simulink model "TECM_SeriesParallel"  (R2023a)
settings: Solver=daessc  StartTime=0.0  StopTime=20E4
libraries: fl_lib x34, nesl_utility x24, BatteryLibrary_lib x5
settings Model: Creator=widana_d  LastModifiedBy=widana_d
settings SolverCC: SolverResetMethod=Robust
settings DataIOCC: SaveState=on
settings OptimizationCC: ReuseModelBlockBuffer=off
settings DebuggingCC: UnconnectedInputMsg=warning  UnconnectedOutputMsg=warning  UnconnectedLineMsg=warning
settings ModelReferenceCC: EnableRefExpFcnMdlSchedulingChecks=on
settings RTWCC: DLArmComputeVersion=19.05

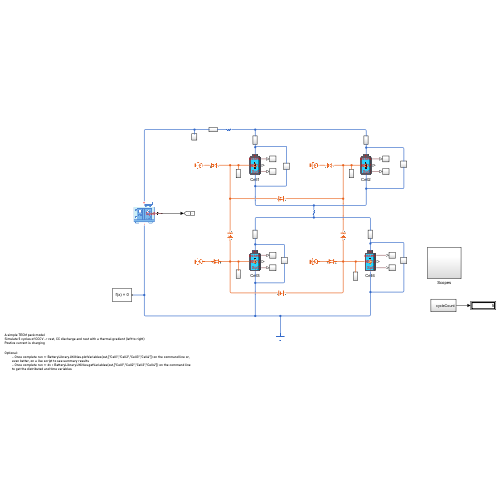
[thumbnail: Simulink's stored preview of the top-level diagram]
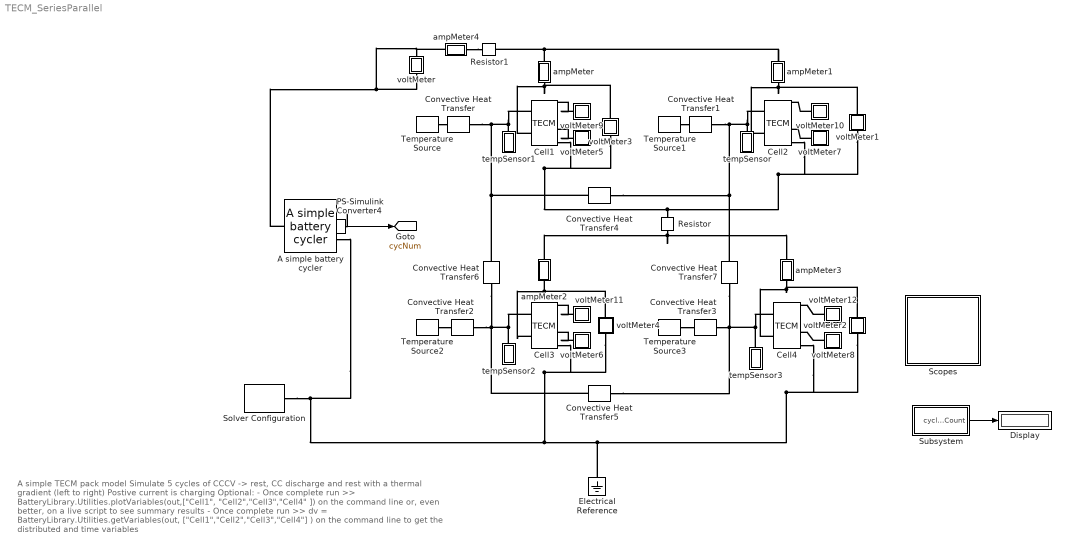
== system TECM_SeriesParallel ==
  note: A simple TECM pack model
      | Simulate 5 cycles of CCCV -> rest, CC discharge and rest with a thermal gradient (left to right)
      | Postive current is charging
      |
      | Optional:
      | - Once complete run >> BatteryLibrary.Utilities.plotVariables(out,["Cell1", "Cell2","Cell3","Cell4" ]) on the command line or, even better, on a live script to see summary results
      | - Once complete run >> dv = BatteryLibrary.Utilities.getVariables(out, ["Cell1","Cell2","Cell3","Cell4"] ) on the command line to get the distributed and time variables
  A simple battery cycler : BatteryLibrary_lib/Utilities/A simple battery cycler  Vmax=8.3 V  Vmin=6.2 V  Ic=4 A  Ico=0.5 A  Id=-10 A  tRestC=1800 s  tRestD=3600 s
      settings: InternalSimscapePortConfiguration="{\"Bottom\":[{\"id\":\"n\",\"label\":\"-\",\"type\":\"foundation.electrical.electrical\"}],\"Left\":[],\"Right\":[{\"id\":\"numCyc\",\"label\":\"Cyc#\",\"type\":\"output\"}],\"Top\":[{\"id\":\"p\",\"label\":\"+\",\"type\":\"foundation.electrical.electrical\"}]}"
  Cell{1..4} (4 alike) : BatteryLibrary_lib/Models/TECM  z0=0.2  T0=298 K  Cn=4.0 A*hr  RoLUT=[.116, .097, .0979, .111; .079, .0617, .0636, .0708; .0526, .0424, .0438, .0483; .0339, .0314, .0325, .0338] Ohm  RpLUT=[.153, .035, .0738, .051; .043, .0323, .0532, .0401; .0293, .0197, .0357, .021; .0124, .00855, .0183, .00974] Ohm  TauLUT=[3.42, 38.3, 66.8, 38.5; 3.19, 46.9, 59.6, 37.5; 47.1, 41.3, 63.9, 32; 23.2, 19.6, 41.2, 16.1] s  tempLUT=[273, 283, 298, 318] K  socLUT=[20.79, 50.5, 80.2, 95.05]/100  Cp=100 J/K  refSoC=[0 : 100]' / 100  refOCV=[3.32, 3.33, 3.34, 3.35, 3.35, 3.36, 3.38, 3.39, 3.4, 3.42, 3.43, 3.44, 3.45, 3.46, 3.47, 3.48, 3.49, 3.5, 3.51, 3.52, 3.52, 3.53, 3.54, 3.54, 3.55, 3.55, 3.56, 3.56, 3.57, 3.57, 3.58, 3.58, 3.59, 3.59, 3.6, 3.6, 3.61, 3.61, 3.62, 3.62, 3.63, 3.63, 3.64, 3.64, 3.65, 3.65, 3.66, 3.67, 3.68, 3.69, 3.7, 3.71, 3.72, 3.74, 3.75, 3.76, 3.76, 3.77, 3.78, 3.79, 3.8, 3.81, 3.81, 3.82, 3.83, 3.84, 3.85, 3.85, 3.86, 3.87, 3.88, 3.88, 3.89, 3.9, 3.9, 3.91, 3.92, 3.93, 3.94, 3.94, 3.95, 3.96, 3.97, 3.98, 3.99, 4, 4.01, 4.02, 4.03, 4.04, 4.05, 4.06, 4.07, 4.08, 4.09, 4.1, 4.11, 4.12, 4.13, 4.14, 4.15]' V
      settings: InternalSimscapePortConfiguration="{\"Bottom\":[{\"id\":\"n\",\"label\":\"-\",\"type\":\"foundation.electrical.electrical\"}],\"Left\":[{\"id\":\"Hi\",\"label\":\"H\",\"type\":\"foundation.thermal.thermal\"}],\"Right\":[{\"id\":\"eta\",\"label\":\"Losses\",\"type\":\"output\"},{\"id\":\"OCV\",\"label\":\"OCV\",\"type\":\"output\"},{\"id\":\"z\",\"label\":\"SoC\",\"type\":\"output\"}],\"Top\":[{\"id\":\"p\",\"label\":\"+\",\"type\":\"foundation.electrical.electrical\"}]}"
  Convective Heat Transfer{,1..3} (4 alike) : fl_lib/Thermal/Thermal Elements/Convective Heat Transfer  thermal_type=foundation.enum.constant_variable.constant  area=0.0023 m^2  heat_tr_coeff=35 W/(m^2 * K)  min_heat_tr_coeff=1e-3 W/(K*m^2)  T_specify=off  T_priority=None  T=0 K  T_nominal_specify=off  T_nominal_unit=K  T_nominal_value=1  Q_specify=off  Q_priority=None  Q=0 W  Q_nominal_specify=off  Q_nominal_unit=W  Q_nominal_value=1
  Convective Heat Transfer4 : fl_lib/Thermal/Thermal Elements/Convective Heat Transfer  thermal_type=foundation.enum.constant_variable.constant  area=0.0015 m^2  heat_tr_coeff=10 W/(m^2 * K)  min_heat_tr_coeff=1e-3 W/(K*m^2)  T_specify=off  T_priority=None  T=0 K  T_nominal_specify=off  T_nominal_unit=K  T_nominal_value=1  Q_specify=off  Q_priority=None  Q=0 W  Q_nominal_specify=off  Q_nominal_unit=W  Q_nominal_value=1
  Convective Heat Transfer5 : fl_lib/Thermal/Thermal Elements/Convective Heat Transfer  thermal_type=foundation.enum.constant_variable.constant  area=0.00115 m^2  heat_tr_coeff=10 W/(m^2 * K)  min_heat_tr_coeff=1e-3 W/(K*m^2)  T_specify=off  T_priority=None  T=0 K  T_nominal_specify=off  T_nominal_unit=K  T_nominal_value=1  Q_specify=off  Q_priority=None  Q=0 W  Q_nominal_specify=off  Q_nominal_unit=W  Q_nominal_value=1
  Convective Heat Transfer6 : fl_lib/Thermal/Thermal Elements/Convective Heat Transfer  thermal_type=foundation.enum.constant_variable.constant  area=0.00115 m^2  heat_tr_coeff=10 W/(m^2 * K)  min_heat_tr_coeff=1e-3 W/(K*m^2)  T_specify=off  T_priority=None  T=0 K  T_nominal_specify=off  T_nominal_unit=K  T_nominal_value=1  Q_specify=off  Q_priority=None  Q=0 W  Q_nominal_specify=off  Q_nominal_unit=W  Q_nominal_value=1
  Convective Heat Transfer7 : fl_lib/Thermal/Thermal Elements/Convective Heat Transfer  thermal_type=foundation.enum.constant_variable.constant  area=0.00115 m^2  heat_tr_coeff=10 W/(m^2 * K)  min_heat_tr_coeff=1e-3 W/(K*m^2)  T_specify=off  T_priority=None  T=0 K  T_nominal_specify=off  T_nominal_unit=K  T_nominal_value=1  Q_specify=off  Q_priority=None  Q=0 W  Q_nominal_specify=off  Q_nominal_unit=W  Q_nominal_value=1
  Display : Display
  Electrical Reference : fl_lib/Electrical/Electrical Elements/Electrical Reference
  PS-Simulink Converter4 : nesl_utility/PS-Simulink Converter  PhysicalDomain=network_engine_domain  SubClassName=ps_output  LeftPortType=input  RightPortType=output  PseudoPeriodic=off  Frequencies=[]  VectorFormat=1-D array  Unit=inherit  AffineConversion=off
  Resistor : fl_lib/Electrical/Electrical Elements/Resistor  R=1e-3 Ohm  i_specify=off  i_priority=None  i=0 A  i_nominal_specify=off  i_nominal_unit=A  i_nominal_value=1  v_specify=off  v_priority=None  v=0 V  v_nominal_specify=off  v_nominal_unit=V  v_nominal_value=1
  Resistor1 : fl_lib/Electrical/Electrical Elements/Resistor  R=1e-3 Ohm  i_specify=off  i_priority=None  i=0 A  i_nominal_specify=off  i_nominal_unit=A  i_nominal_value=1  v_specify=off  v_priority=None  v=0 V  v_nominal_specify=off  v_nominal_unit=V  v_nominal_value=1
  Scopes : Subsystem
  Solver Configuration : nesl_utility/Solver Configuration  PhysicalDomain=network_engine_domain  SubClassName=solver  LeftPortType=input  RightPortType=generic  Tones=[]  Harmonics=[]  SimulateNoise=off  Profile=off  UseLocalSampling=off  EnableSwitchedLinearOptims=on  FrequencyDomain=off  UseCCode=off  RelTol=0.001  AbsTol=1e-06  MinStep=1e-09  ToWorkspace=off  RevertToSquareIcSolve=off  NumHomotopyIterations=100  PhasorMode=off  PhasorModeNumHarmonics=1  ConsistencySolver=NEWTON_FTOL  IndexReductionMethod=DerivativeReplacement  DoDC=off  ResidualTolerance=1e-09  ConsistencyTolSource=GLOBAL  ConsistencyAbsTol=0.001  ConsistencyRelTol=0.001  ConsistencyTolFactor=0.001  UseLocalSolver=off  LocalSolverChoice=NE_BACKWARD_EULER_ADVANCER  ResolveIndetEquations=on  FunctionEvalNumThread=1  LocalSolverSampleTime=0.001  DoFixedCost=off  MaxNonlinIter=3  MaxModeIter=2  ComputeImpulses=off  ImpulseIterations=2  LinearAlgebra=auto  LinearAlgebraNumThread=0  EquationFormulation=NE_TIME_EF  DelaysMemoryBudget=1024  AutomaticFiltering=on  FilteringTimeConstant=0.001  PartitionStorageMethod=AS_NEEDED  PartitionMemoryBudget=1024  PartitionMethod=ROBUST
  Subsystem : Subsystem
  Temperature Source : fl_lib/Thermal/Thermal Sources/Temperature Source  temperature=20 degC
  Temperature Source1 : fl_lib/Thermal/Thermal Sources/Temperature Source  temperature=30 degC
  Temperature Source2 : fl_lib/Thermal/Thermal Sources/Temperature Source  temperature=20 degC
  Temperature Source3 : fl_lib/Thermal/Thermal Sources/Temperature Source  temperature=30 degC
  ampMeter : Subsystem
  ampMeter1 : Subsystem
  ampMeter2 : Subsystem
  ampMeter3 : Subsystem
  ampMeter4 : Subsystem
  tempSensor : Subsystem
  tempSensor1 : Subsystem
  tempSensor2 : Subsystem
  tempSensor3 : Subsystem
  voltMeter : Subsystem
  voltMeter1 : Subsystem
  voltMeter10 : Subsystem
  voltMeter11 : Subsystem
  voltMeter12 : Subsystem
  voltMeter2 : Subsystem
  voltMeter3 : Subsystem
  voltMeter4 : Subsystem
  voltMeter5 : Subsystem
  voltMeter6 : Subsystem
  voltMeter7 : Subsystem
  voltMeter8 : Subsystem
  voltMeter9 : Subsystem
  tag scope: cycNum=global
  wires:
  Subsystem/1(cycleCount) -> Display/1
  PS-Simulink Converter4/1 -> [cycNum]
  connections:
  ampMeter/LConn1 -- ampMeter1/LConn1 -- Resistor1/RConn1
  voltMeter4/RConn1 -- Cell3/RConn4 -- A simple battery cycler/RConn2 -- Solver Configuration/RConn1 -- Cell4/RConn4 -- voltMeter2/RConn1 -- Electrical Reference/LConn1
  ampMeter2/LConn1 -- Resistor/LConn1 -- ampMeter3/LConn1
  ampMeter/RConn1 -- Cell1/LConn2 -- voltMeter3/LConn1
  ampMeter1/RConn1 -- Cell2/LConn2 -- voltMeter1/LConn1
  voltMeter4/LConn1 -- Cell3/LConn2 -- ampMeter2/RConn1
  ampMeter3/RConn1 -- Cell4/LConn2 -- voltMeter2/LConn1
  Convective Heat Transfer/LConn1 -- Convective Heat Transfer6/LConn1 -- Convective Heat Transfer4/RConn1 -- Cell1/LConn1 -- tempSensor1/LConn1
  Convective Heat Transfer1/LConn1 -- Convective Heat Transfer4/LConn1 -- Convective Heat Transfer7/LConn1 -- Cell2/LConn1 -- tempSensor/LConn1
  Convective Heat Transfer2/LConn1 -- Convective Heat Transfer6/RConn1 -- Cell3/LConn1 -- tempSensor2/LConn1 -- Convective Heat Transfer5/RConn1
  Convective Heat Transfer3/LConn1 -- Cell4/LConn1 -- tempSensor3/LConn1 -- Convective Heat Transfer5/LConn1 -- Convective Heat Transfer7/RConn1
  Temperature Source/LConn1 -- Convective Heat Transfer/RConn1
  Temperature Source1/LConn1 -- Convective Heat Transfer1/RConn1
  voltMeter3/RConn1 -- Cell1/RConn4 -- Resistor/RConn1 -- Cell2/RConn4 -- voltMeter1/RConn1
  A simple battery cycler/LConn1 -- ampMeter4/LConn1 -- voltMeter/LConn1
  Temperature Source2/LConn1 -- Convective Heat Transfer2/RConn1
  Temperature Source3/LConn1 -- Convective Heat Transfer3/RConn1
  PS-Simulink Converter4/LConn1 -- A simple battery cycler/RConn1
  voltMeter9/LConn1 -- Cell1/RConn1
  voltMeter11/LConn1 -- Cell3/RConn1
  voltMeter10/LConn1 -- Cell2/RConn1
  voltMeter12/LConn1 -- Cell4/RConn1
  voltMeter5/LConn1 -- Cell1/RConn3
  voltMeter7/LConn1 -- Cell2/RConn3
  voltMeter6/LConn1 -- Cell3/RConn3
  voltMeter8/LConn1 -- Cell4/RConn3
  ampMeter4/RConn1 -- Resistor1/LConn1

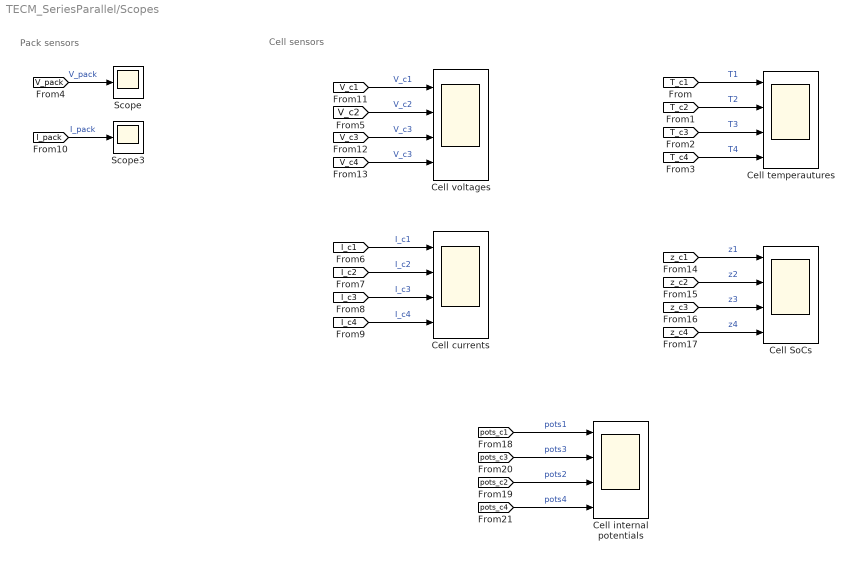
== system TECM_SeriesParallel/Scopes ==
  note: Cell sensors
  note: Pack sensors
  Cell SoCs : Scope  NumInputPorts=4
  Cell currents : Scope  NumInputPorts=4
  Cell internal potentials : Scope  NumInputPorts=4
  Cell temperautures : Scope  NumInputPorts=4
  Cell voltages : Scope  NumInputPorts=4
  Scope : Scope
  Scope3 : Scope
  wires:
  [I_c2] -> Cell currents/2  "I_c2"
  [V_c1] -> Cell voltages/1  "V_c1"
  [I_pack] -> Scope3/1  "I_pack"
  [I_c3] -> Cell currents/3  "I_c3"
  [V_c2] -> Cell voltages/2  "V_c2"
  [V_c4] -> Cell voltages/4  "V_c3"
  [V_pack] -> Scope/1  "V_pack"
  [V_c3] -> Cell voltages/3  "V_c3"
  [I_c4] -> Cell currents/4  "I_c4"
  [I_c1] -> Cell currents/1  "I_c1"
  [T_c2] -> Cell temperautures/2  "T2"
  [T_c1] -> Cell temperautures/1  "T1"
  [T_c3] -> Cell temperautures/3  "T3"
  [T_c4] -> Cell temperautures/4  "T4"
  [z_c3] -> Cell SoCs/3  "z3"
  [z_c4] -> Cell SoCs/4  "z4"
  [z_c1] -> Cell SoCs/1  "z1"
  [z_c2] -> Cell SoCs/2  "z2"
  [pots_c2] -> Cell internal potentials/3  "pots2"
  [pots_c1] -> Cell internal potentials/1  "pots1"
  [pots_c4] -> Cell internal potentials/4  "pots4"
  [pots_c3] -> Cell internal potentials/2  "pots3"

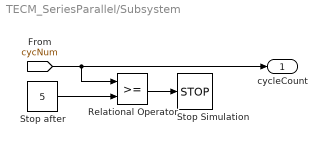
== system TECM_SeriesParallel/Subsystem ==
  Relational Operator : RelationalOperator  OutDataTypeStr=boolean  RndMeth=Simplest  InputSameDT=off
  Stop Simulation : Stop
  Stop after : Constant  Value=5
  cycleCount : Outport
  wires:
  Stop after/1 -> Relational Operator/2
  [cycNum] -> cycleCount/1, Relational Operator/1
  Relational Operator/1 -> Stop Simulation/1

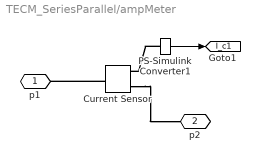
== system TECM_SeriesParallel/ampMeter ==
  Current Sensor : fl_lib/Electrical/Electrical Sensors/Current Sensor
  PS-Simulink Converter1 : nesl_utility/PS-Simulink Converter  PhysicalDomain=network_engine_domain  SubClassName=ps_output  LeftPortType=input  RightPortType=output  PseudoPeriodic=off  Frequencies=[]  VectorFormat=1-D array  Unit=inherit  AffineConversion=off
  p1 : PMIOPort  Side=Left
  p2 : PMIOPort  Port=2  Side=Right
  tag scope: I_c1=global
  wires:
  PS-Simulink Converter1/1 -> [I_c1]
  connections:
  Current Sensor/RConn2 -- p2/RConn1
  Current Sensor/LConn1 -- p1/RConn1
  PS-Simulink Converter1/LConn1 -- Current Sensor/RConn1

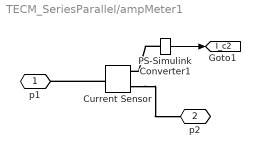
== system TECM_SeriesParallel/ampMeter1 ==
  Current Sensor : fl_lib/Electrical/Electrical Sensors/Current Sensor
  PS-Simulink Converter1 : nesl_utility/PS-Simulink Converter  PhysicalDomain=network_engine_domain  SubClassName=ps_output  LeftPortType=input  RightPortType=output  PseudoPeriodic=off  Frequencies=[]  VectorFormat=1-D array  Unit=inherit  AffineConversion=off
  p1 : PMIOPort  Side=Left
  p2 : PMIOPort  Port=2  Side=Right
  tag scope: I_c2=global
  wires:
  PS-Simulink Converter1/1 -> [I_c2]
  connections:
  Current Sensor/RConn2 -- p2/RConn1
  Current Sensor/LConn1 -- p1/RConn1
  PS-Simulink Converter1/LConn1 -- Current Sensor/RConn1

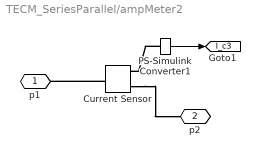
== system TECM_SeriesParallel/ampMeter2 ==
  Current Sensor : fl_lib/Electrical/Electrical Sensors/Current Sensor
  PS-Simulink Converter1 : nesl_utility/PS-Simulink Converter  PhysicalDomain=network_engine_domain  SubClassName=ps_output  LeftPortType=input  RightPortType=output  PseudoPeriodic=off  Frequencies=[]  VectorFormat=1-D array  Unit=inherit  AffineConversion=off
  p1 : PMIOPort  Side=Left
  p2 : PMIOPort  Port=2  Side=Right
  tag scope: I_c3=global
  wires:
  PS-Simulink Converter1/1 -> [I_c3]
  connections:
  Current Sensor/RConn2 -- p2/RConn1
  Current Sensor/LConn1 -- p1/RConn1
  PS-Simulink Converter1/LConn1 -- Current Sensor/RConn1

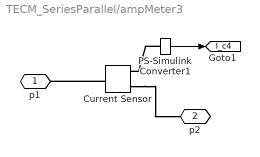
== system TECM_SeriesParallel/ampMeter3 ==
  Current Sensor : fl_lib/Electrical/Electrical Sensors/Current Sensor
  PS-Simulink Converter1 : nesl_utility/PS-Simulink Converter  PhysicalDomain=network_engine_domain  SubClassName=ps_output  LeftPortType=input  RightPortType=output  PseudoPeriodic=off  Frequencies=[]  VectorFormat=1-D array  Unit=inherit  AffineConversion=off
  p1 : PMIOPort  Side=Left
  p2 : PMIOPort  Port=2  Side=Right
  tag scope: I_c4=global
  wires:
  PS-Simulink Converter1/1 -> [I_c4]
  connections:
  Current Sensor/RConn2 -- p2/RConn1
  Current Sensor/LConn1 -- p1/RConn1
  PS-Simulink Converter1/LConn1 -- Current Sensor/RConn1

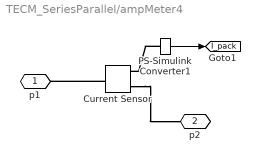
== system TECM_SeriesParallel/ampMeter4 ==
  Current Sensor : fl_lib/Electrical/Electrical Sensors/Current Sensor
  PS-Simulink Converter1 : nesl_utility/PS-Simulink Converter  PhysicalDomain=network_engine_domain  SubClassName=ps_output  LeftPortType=input  RightPortType=output  PseudoPeriodic=off  Frequencies=[]  VectorFormat=1-D array  Unit=inherit  AffineConversion=off
  p1 : PMIOPort  Side=Left
  p2 : PMIOPort  Port=2  Side=Right
  tag scope: I_pack=global
  wires:
  PS-Simulink Converter1/1 -> [I_pack]
  connections:
  Current Sensor/RConn2 -- p2/RConn1
  Current Sensor/LConn1 -- p1/RConn1
  PS-Simulink Converter1/LConn1 -- Current Sensor/RConn1

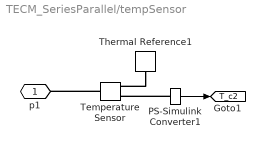
== system TECM_SeriesParallel/tempSensor ==
  PS-Simulink Converter1 : nesl_utility/PS-Simulink Converter  PhysicalDomain=network_engine_domain  SubClassName=ps_output  LeftPortType=input  RightPortType=output  PseudoPeriodic=off  Frequencies=[]  VectorFormat=1-D array  Unit=inherit  AffineConversion=off
  Temperature Sensor : fl_lib/Thermal/Thermal Sensors/Temperature Sensor  temperature_measure=foundation.enum.MeasurementReference.difference
  Thermal Reference1 : fl_lib/Thermal/Thermal Elements/Thermal Reference
  p1 : PMIOPort  Side=Left
  tag scope: T_c2=global
  wires:
  PS-Simulink Converter1/1 -> [T_c2]
  connections:
  Temperature Sensor/LConn1 -- p1/RConn1
  PS-Simulink Converter1/LConn1 -- Temperature Sensor/RConn2
  Thermal Reference1/LConn1 -- Temperature Sensor/RConn1

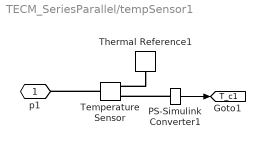
== system TECM_SeriesParallel/tempSensor1 ==
  PS-Simulink Converter1 : nesl_utility/PS-Simulink Converter  PhysicalDomain=network_engine_domain  SubClassName=ps_output  LeftPortType=input  RightPortType=output  PseudoPeriodic=off  Frequencies=[]  VectorFormat=1-D array  Unit=inherit  AffineConversion=off
  Temperature Sensor : fl_lib/Thermal/Thermal Sensors/Temperature Sensor  temperature_measure=foundation.enum.MeasurementReference.difference
  Thermal Reference1 : fl_lib/Thermal/Thermal Elements/Thermal Reference
  p1 : PMIOPort  Side=Left
  tag scope: T_c1=global
  wires:
  PS-Simulink Converter1/1 -> [T_c1]
  connections:
  Temperature Sensor/LConn1 -- p1/RConn1
  PS-Simulink Converter1/LConn1 -- Temperature Sensor/RConn2
  Thermal Reference1/LConn1 -- Temperature Sensor/RConn1

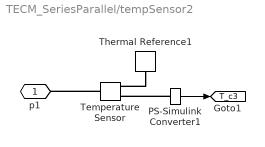
== system TECM_SeriesParallel/tempSensor2 ==
  PS-Simulink Converter1 : nesl_utility/PS-Simulink Converter  PhysicalDomain=network_engine_domain  SubClassName=ps_output  LeftPortType=input  RightPortType=output  PseudoPeriodic=off  Frequencies=[]  VectorFormat=1-D array  Unit=inherit  AffineConversion=off
  Temperature Sensor : fl_lib/Thermal/Thermal Sensors/Temperature Sensor  temperature_measure=foundation.enum.MeasurementReference.difference
  Thermal Reference1 : fl_lib/Thermal/Thermal Elements/Thermal Reference
  p1 : PMIOPort  Side=Left
  tag scope: T_c3=global
  wires:
  PS-Simulink Converter1/1 -> [T_c3]
  connections:
  Temperature Sensor/LConn1 -- p1/RConn1
  PS-Simulink Converter1/LConn1 -- Temperature Sensor/RConn2
  Thermal Reference1/LConn1 -- Temperature Sensor/RConn1

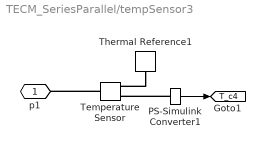
== system TECM_SeriesParallel/tempSensor3 ==
  PS-Simulink Converter1 : nesl_utility/PS-Simulink Converter  PhysicalDomain=network_engine_domain  SubClassName=ps_output  LeftPortType=input  RightPortType=output  PseudoPeriodic=off  Frequencies=[]  VectorFormat=1-D array  Unit=inherit  AffineConversion=off
  Temperature Sensor : fl_lib/Thermal/Thermal Sensors/Temperature Sensor  temperature_measure=foundation.enum.MeasurementReference.difference
  Thermal Reference1 : fl_lib/Thermal/Thermal Elements/Thermal Reference
  p1 : PMIOPort  Side=Left
  tag scope: T_c4=global
  wires:
  PS-Simulink Converter1/1 -> [T_c4]
  connections:
  Temperature Sensor/LConn1 -- p1/RConn1
  PS-Simulink Converter1/LConn1 -- Temperature Sensor/RConn2
  Thermal Reference1/LConn1 -- Temperature Sensor/RConn1

== system TECM_SeriesParallel/voltMeter ==
  Electrical Reference1 : fl_lib/Electrical/Electrical Elements/Electrical Reference
  PS-Simulink Converter : nesl_utility/PS-Simulink Converter  PhysicalDomain=network_engine_domain  SubClassName=ps_output  LeftPortType=input  RightPortType=output  PseudoPeriodic=off  Frequencies=[]  VectorFormat=1-D array  Unit=inherit  AffineConversion=off
  Voltage Sensor : fl_lib/Electrical/Electrical Sensors/Voltage Sensor
  Conn1 : PMIOPort  Side=Left
  tag scope: V_pack=global
  wires:
  PS-Simulink Converter/1 -> [V_pack]  "V"
  connections:
  Voltage Sensor/LConn1 -- Conn1/RConn1
  PS-Simulink Converter/LConn1 -- Voltage Sensor/RConn1
  Electrical Reference1/LConn1 -- Voltage Sensor/RConn2

== system TECM_SeriesParallel/voltMeter1 ==
  PS-Simulink Converter : nesl_utility/PS-Simulink Converter  PhysicalDomain=network_engine_domain  SubClassName=ps_output  LeftPortType=input  RightPortType=output  PseudoPeriodic=off  Frequencies=[]  VectorFormat=1-D array  Unit=inherit  AffineConversion=off
  Voltage Sensor : fl_lib/Electrical/Electrical Sensors/Voltage Sensor
  p1 : PMIOPort  Side=Left
  p2 : PMIOPort  Port=2  Side=Right
  tag scope: V_c2=global
  wires:
  PS-Simulink Converter/1 -> [V_c2]  "V"
  connections:
  Voltage Sensor/LConn1 -- p1/RConn1
  PS-Simulink Converter/LConn1 -- Voltage Sensor/RConn1
  p2/RConn1 -- Voltage Sensor/RConn2

== system TECM_SeriesParallel/voltMeter10 ==
  PS-Simulink Converter : nesl_utility/PS-Simulink Converter  PhysicalDomain=network_engine_domain  SubClassName=ps_output  LeftPortType=input  RightPortType=output  PseudoPeriodic=off  Frequencies=[]  VectorFormat=1-D array  Unit=inherit  AffineConversion=off
  p1 : PMIOPort  Side=Left
  tag scope: pots_c2=global
  wires:
  PS-Simulink Converter/1 -> [pots_c2]  "V"
  connections:
  p1/RConn1 -- PS-Simulink Converter/LConn1

== system TECM_SeriesParallel/voltMeter11 ==
  PS-Simulink Converter : nesl_utility/PS-Simulink Converter  PhysicalDomain=network_engine_domain  SubClassName=ps_output  LeftPortType=input  RightPortType=output  PseudoPeriodic=off  Frequencies=[]  VectorFormat=1-D array  Unit=inherit  AffineConversion=off
  p1 : PMIOPort  Side=Left
  tag scope: pots_c3=global
  wires:
  PS-Simulink Converter/1 -> [pots_c3]  "V"
  connections:
  p1/RConn1 -- PS-Simulink Converter/LConn1

== system TECM_SeriesParallel/voltMeter12 ==
  PS-Simulink Converter : nesl_utility/PS-Simulink Converter  PhysicalDomain=network_engine_domain  SubClassName=ps_output  LeftPortType=input  RightPortType=output  PseudoPeriodic=off  Frequencies=[]  VectorFormat=1-D array  Unit=inherit  AffineConversion=off
  p1 : PMIOPort  Side=Left
  tag scope: pots_c4=global
  wires:
  PS-Simulink Converter/1 -> [pots_c4]  "V"
  connections:
  p1/RConn1 -- PS-Simulink Converter/LConn1

== system TECM_SeriesParallel/voltMeter2 ==
  PS-Simulink Converter : nesl_utility/PS-Simulink Converter  PhysicalDomain=network_engine_domain  SubClassName=ps_output  LeftPortType=input  RightPortType=output  PseudoPeriodic=off  Frequencies=[]  VectorFormat=1-D array  Unit=inherit  AffineConversion=off
  Voltage Sensor : fl_lib/Electrical/Electrical Sensors/Voltage Sensor
  p1 : PMIOPort  Side=Left
  p2 : PMIOPort  Port=2  Side=Right
  tag scope: V_c4=global
  wires:
  PS-Simulink Converter/1 -> [V_c4]  "V"
  connections:
  Voltage Sensor/LConn1 -- p1/RConn1
  PS-Simulink Converter/LConn1 -- Voltage Sensor/RConn1
  p2/RConn1 -- Voltage Sensor/RConn2

== system TECM_SeriesParallel/voltMeter3 ==
  PS-Simulink Converter : nesl_utility/PS-Simulink Converter  PhysicalDomain=network_engine_domain  SubClassName=ps_output  LeftPortType=input  RightPortType=output  PseudoPeriodic=off  Frequencies=[]  VectorFormat=1-D array  Unit=inherit  AffineConversion=off
  Voltage Sensor : fl_lib/Electrical/Electrical Sensors/Voltage Sensor
  p1 : PMIOPort  Side=Left
  p2 : PMIOPort  Port=2  Side=Right
  tag scope: V_c1=global
  wires:
  PS-Simulink Converter/1 -> [V_c1]  "V"
  connections:
  Voltage Sensor/LConn1 -- p1/RConn1
  PS-Simulink Converter/LConn1 -- Voltage Sensor/RConn1
  p2/RConn1 -- Voltage Sensor/RConn2

== system TECM_SeriesParallel/voltMeter4 ==
  PS-Simulink Converter : nesl_utility/PS-Simulink Converter  PhysicalDomain=network_engine_domain  SubClassName=ps_output  LeftPortType=input  RightPortType=output  PseudoPeriodic=off  Frequencies=[]  VectorFormat=1-D array  Unit=inherit  AffineConversion=off
  Voltage Sensor : fl_lib/Electrical/Electrical Sensors/Voltage Sensor
  p1 : PMIOPort  Side=Left
  p2 : PMIOPort  Port=2  Side=Right
  tag scope: V_c3=global
  wires:
  PS-Simulink Converter/1 -> [V_c3]  "V"
  connections:
  Voltage Sensor/LConn1 -- p1/RConn1
  PS-Simulink Converter/LConn1 -- Voltage Sensor/RConn1
  p2/RConn1 -- Voltage Sensor/RConn2

== system TECM_SeriesParallel/voltMeter5 ==
  PS-Simulink Converter : nesl_utility/PS-Simulink Converter  PhysicalDomain=network_engine_domain  SubClassName=ps_output  LeftPortType=input  RightPortType=output  PseudoPeriodic=off  Frequencies=[]  VectorFormat=1-D array  Unit=inherit  AffineConversion=off
  p1 : PMIOPort  Side=Left
  tag scope: z_c1=global
  wires:
  PS-Simulink Converter/1 -> [z_c1]  "V"
  connections:
  p1/RConn1 -- PS-Simulink Converter/LConn1

== system TECM_SeriesParallel/voltMeter6 ==
  PS-Simulink Converter : nesl_utility/PS-Simulink Converter  PhysicalDomain=network_engine_domain  SubClassName=ps_output  LeftPortType=input  RightPortType=output  PseudoPeriodic=off  Frequencies=[]  VectorFormat=1-D array  Unit=inherit  AffineConversion=off
  p1 : PMIOPort  Side=Left
  tag scope: z_c3=global
  wires:
  PS-Simulink Converter/1 -> [z_c3]  "V"
  connections:
  p1/RConn1 -- PS-Simulink Converter/LConn1

== system TECM_SeriesParallel/voltMeter7 ==
  PS-Simulink Converter : nesl_utility/PS-Simulink Converter  PhysicalDomain=network_engine_domain  SubClassName=ps_output  LeftPortType=input  RightPortType=output  PseudoPeriodic=off  Frequencies=[]  VectorFormat=1-D array  Unit=inherit  AffineConversion=off
  p1 : PMIOPort  Side=Left
  tag scope: z_c2=global
  wires:
  PS-Simulink Converter/1 -> [z_c2]  "V"
  connections:
  p1/RConn1 -- PS-Simulink Converter/LConn1

== system TECM_SeriesParallel/voltMeter8 ==
  PS-Simulink Converter : nesl_utility/PS-Simulink Converter  PhysicalDomain=network_engine_domain  SubClassName=ps_output  LeftPortType=input  RightPortType=output  PseudoPeriodic=off  Frequencies=[]  VectorFormat=1-D array  Unit=inherit  AffineConversion=off
  p1 : PMIOPort  Side=Left
  tag scope: z_c4=global
  wires:
  PS-Simulink Converter/1 -> [z_c4]  "V"
  connections:
  p1/RConn1 -- PS-Simulink Converter/LConn1

== system TECM_SeriesParallel/voltMeter9 ==
  PS-Simulink Converter : nesl_utility/PS-Simulink Converter  PhysicalDomain=network_engine_domain  SubClassName=ps_output  LeftPortType=input  RightPortType=output  PseudoPeriodic=off  Frequencies=[]  VectorFormat=1-D array  Unit=inherit  AffineConversion=off
  p1 : PMIOPort  Side=Left
  tag scope: pots_c1=global
  wires:
  PS-Simulink Converter/1 -> [pots_c1]  "V"
  connections:
  p1/RConn1 -- PS-Simulink Converter/LConn1
